simulink model "maglev_cl_sim"  (R2026a)
settings: Solver=ode4  StopTime=sc.Tend  FixedStep=L.T0/10
undefined symbols (not defined in the file or in its folder): C, DiscIntNeverNeededParam, L, pl, sc
libraries: simulink x1
Description:
  | [STANDALONE] Closed-loop MagLev simulation (nonlinear plant + lab cascade controller). Built by scripts/build_maglev_cl_sim.m. Parameters: workspace structs pl, C, L, sc (see scripts/maglev_cases.m).
settings Model: Creator=gargr  LastModifiedBy=gargr
settings DebuggingCC: AlgebraicLoopMsg=error

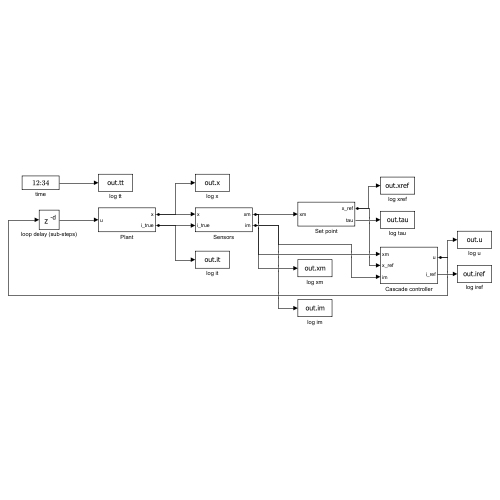
[thumbnail: Simulink's stored preview of the top-level diagram]
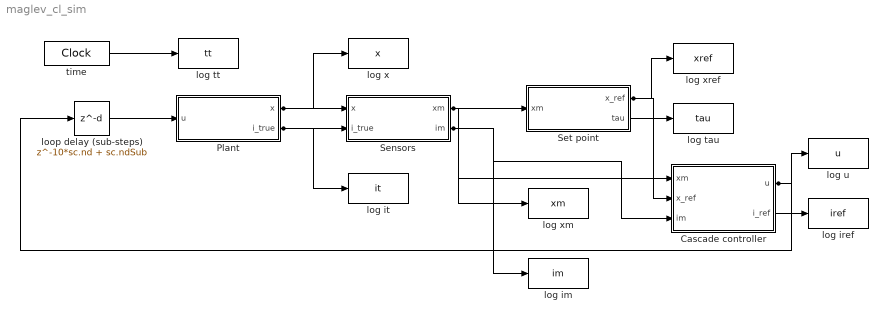
== system maglev_cl_sim ==
  Cascade controller : Subsystem
  Plant : Subsystem
  Sensors : Subsystem
  Set point : Subsystem
  log im : ToWorkspace  VariableName=im  SampleTime=L.T0
  log iref : ToWorkspace  VariableName=iref  SampleTime=L.T0
  log it : ToWorkspace  VariableName=it  SampleTime=L.T0
  log tau : ToWorkspace  VariableName=tau  SampleTime=L.T0
  log tt : ToWorkspace  VariableName=tt  SampleTime=L.T0
  log u : ToWorkspace  VariableName=u  SampleTime=L.T0
  log x : ToWorkspace  VariableName=x  SampleTime=L.T0
  log xm : ToWorkspace  VariableName=xm  SampleTime=L.T0
  log xref : ToWorkspace  VariableName=xref  SampleTime=L.T0
  loop delay (sub-steps) : Delay  DelayLength=10*sc.nd + sc.ndSub  InitialCondition=sc.uIC  SampleTime=L.T0/10
  time : DigitalClock  SampleTime=L.T0
  wires:
  Sensors/2(im) -> Cascade controller/3(im), log im/1
  Sensors/1(xm) -> Set point/1(xm), Cascade controller/1(xm), log xm/1
  time/1 -> log tt/1
  loop delay (sub-steps)/1 -> Plant/1(u)
  Set point/2(tau) -> log tau/1
  Plant/2(i_true) -> Sensors/2(i_true), log it/1
  Plant/1(x) -> Sensors/1(x), log x/1
  Set point/1(x_ref) -> Cascade controller/2(x_ref), log xref/1
  Cascade controller/1(u) -> loop delay (sub-steps)/1, log u/1
  Cascade controller/2(i_ref) -> log iref/1

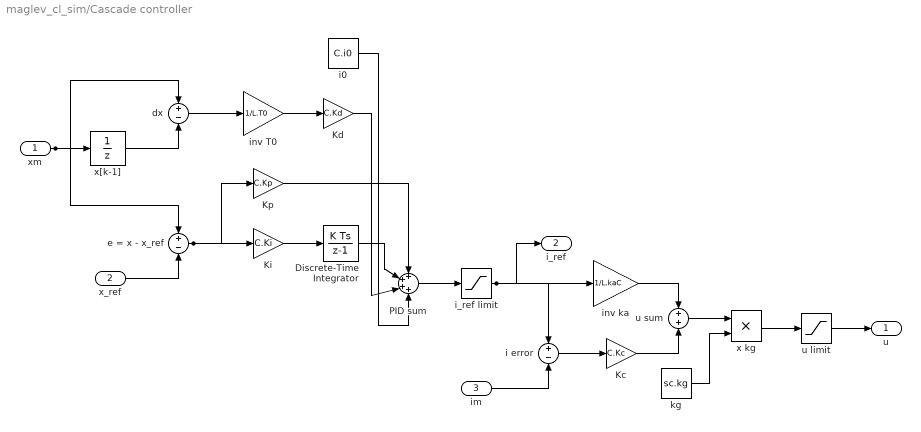
== system maglev_cl_sim/Cascade controller ==
  xm : Inport
  x_ref : Inport  Port=2
  im : Inport  Port=3
  Discrete-Time Integrator : DiscreteIntegrator  InitialCondition=sc.zI  SampleTime=L.T0  LimitOutput=on  UpperSaturationLimit=C.iLim  LowerSaturationLimit=-C.iLim  ICPrevOutput=DiscIntNeverNeededParam  ICPrevScaledInput=DiscIntNeverNeededParam
  Kc : Gain  Gain=C.Kc
  Kd : Gain  Gain=C.Kd
  Ki : Gain  Gain=C.Ki
  Kp : Gain  Gain=C.Kp
  PID sum : Sum  Inputs=++++
  dx : Sum  Inputs=+-
  e = x - x_ref : Sum  Inputs=+-
  i error : Sum  Inputs=+-
  i0 : Constant  Value=C.i0
  i_ref limit : Saturate  UpperLimit=2.0  LowerLimit=0
  inv T0 : Gain  Gain=1/L.T0
  inv ka : Gain  Gain=1/L.kaC
  kg : Constant  Value=sc.kg
  u limit : Saturate  UpperLimit=L.umax  LowerLimit=0
  u sum : Sum
  x kg : Product
  x[k-1] : UnitDelay  InitialCondition=sc.x0  SampleTime=L.T0
  u : Outport
  i_ref : Outport  Port=2
  wires:
  i0/1 -> PID sum/4
  Ki/1 -> Discrete-Time Integrator/1
  i error/1 -> Kc/1
  xm/1 -> e = x - x_ref/1, dx/1, x[k-1]/1
  Kp/1 -> PID sum/1
  inv T0/1 -> Kd/1
  dx/1 -> inv T0/1
  x_ref/1 -> e = x - x_ref/2
  e = x - x_ref/1 -> Kp/1, Ki/1
  x[k-1]/1 -> dx/2
  Kd/1 -> PID sum/3
  Discrete-Time Integrator/1 -> PID sum/2
  PID sum/1 -> i_ref limit/1
  i_ref limit/1 -> i error/1, inv ka/1, i_ref/1
  im/1 -> i error/2
  inv ka/1 -> u sum/1
  u limit/1 -> u/1
  Kc/1 -> u sum/2
  u sum/1 -> x kg/1
  kg/1 -> x kg/2
  x kg/1 -> u limit/1

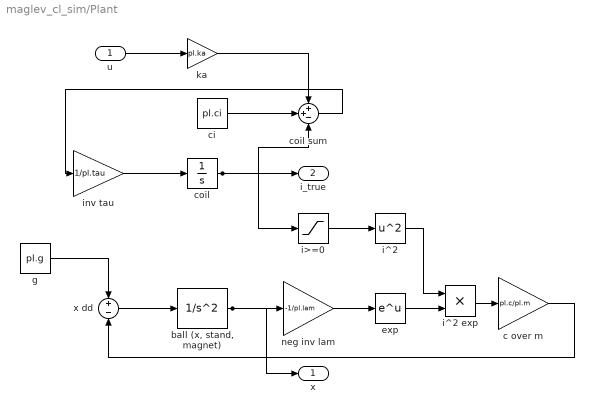
== system maglev_cl_sim/Plant ==
  u : Inport
  "ball (x, stand, magnet)" : SecondOrderIntegrator  ICX=sc.x0  LimitX=on  UpperLimitX=pl.xStand  LowerLimitX=0  ICDXDT=0  ShowOutput=x
  c over m : Gain  Gain=pl.c/pl.m
  ci : Constant  Value=pl.ci
  coil : Integrator  InitialCondition=sc.i0s
  coil sum : Sum  Inputs=++-
  exp : Math
  g : Constant  Value=pl.g
  i>=0 : Saturate  UpperLimit=inf  LowerLimit=0
  i^2 : Math  Operator=square
  i^2 exp : Product
  inv tau : Gain  Gain=1/pl.tau
  ka : Gain  Gain=pl.ka
  neg inv lam : Gain  Gain=-1/pl.lam
  x dd : Sum  Inputs=+-
  x : Outport
  i_true : Outport  Port=2
  wires:
  "ball (x, stand, magnet)"/1 -> neg inv lam/1, x/1
  g/1 -> x dd/1
  x dd/1 -> "ball (x, stand, magnet)"/1
  u/1 -> ka/1
  inv tau/1 -> coil/1
  ka/1 -> coil sum/1
  coil sum/1 -> inv tau/1
  ci/1 -> coil sum/2
  i^2/1 -> i^2 exp/1
  coil/1 -> i_true/1, i>=0/1, coil sum/3
  i>=0/1 -> i^2/1
  neg inv lam/1 -> exp/1
  i^2 exp/1 -> c over m/1
  exp/1 -> i^2 exp/2
  c over m/1 -> x dd/2

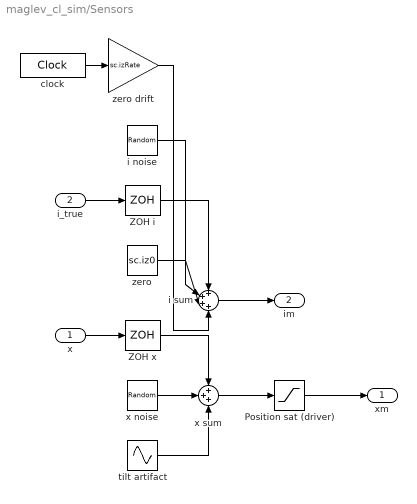
== system maglev_cl_sim/Sensors ==
  x : Inport
  i_true : Inport  Port=2
  Position sat (driver) : Saturate  UpperLimit=0.02  LowerLimit=0
  ZOH i : ZeroOrderHold  SampleTime=L.T0
  ZOH x : ZeroOrderHold  SampleTime=L.T0
  clock : DigitalClock  SampleTime=L.T0
  i noise : RandomNumber  Variance=sc.sigI^2  Seed=sc.seedI  SampleTime=L.T0
  i sum : Sum  Inputs=++++
  tilt artifact : Sin  Amplitude=sc.dxA  Frequency=2*pi*sc.dxF  SampleTime=L.T0
  x noise : RandomNumber  Variance=sc.sigX^2  Seed=sc.seedX  SampleTime=L.T0
  x sum : Sum  Inputs=+++
  zero : Constant  Value=sc.iz0
  zero drift : Gain  Gain=sc.izRate
  xm : Outport
  im : Outport  Port=2
  wires:
  tilt artifact/1 -> x sum/3
  clock/1 -> zero drift/1
  i noise/1 -> i sum/2
  zero drift/1 -> i sum/4
  x/1 -> ZOH x/1
  i_true/1 -> ZOH i/1
  ZOH x/1 -> x sum/1
  ZOH i/1 -> i sum/1
  zero/1 -> i sum/3
  x noise/1 -> x sum/2
  i sum/1 -> im/1
  x sum/1 -> Position sat (driver)/1
  Position sat (driver)/1 -> xm/1

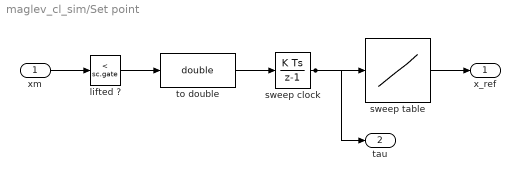
== system maglev_cl_sim/Set point ==
  xm : Inport
  lifted ? : simulink/Logic and Bit Operations/Compare To Constant  relop=<  const=sc.gate  OutDataTypeStr=boolean
  sweep clock : DiscreteIntegrator  SampleTime=L.T0  ICPrevOutput=DiscIntNeverNeededParam  ICPrevScaledInput=DiscIntNeverNeededParam
  sweep table : Lookup_n-D  NumberOfTableDimensions=1  BreakpointsForDimension1=sc.bpT  Table=sc.bpX  InterpMethod=Flat  ExtrapMethod=Clip  InternalRulePriority=Speed  RndMeth=Simplest
  to double : DataTypeConversion  OutDataTypeStr=double  SaturateOnIntegerOverflow=off  RndMeth=Floor
  x_ref : Outport
  tau : Outport  Port=2
  wires:
  xm/1 -> lifted ?/1
  sweep clock/1 -> sweep table/1, tau/1
  to double/1 -> sweep clock/1
  lifted ?/1 -> to double/1
  sweep table/1 -> x_ref/1
